simulink model "sfReuseStates"  (R2025b)
settings: Solver=FixedStepDiscrete  StartTime=0.0  StopTime=10.0  FixedStep=1  RelTol=1e-3  EnableMultiTasking=on
settings Model: Creator=The MathWorks, Inc.  LastModifiedBy=The MathWorks, Inc.
settings SolverCC: AlgebraicLoopSolver=TrustRegion
settings DataIOCC: LimitDataPoints=on  SaveFormat=Array  ReturnWorkspaceOutputs=off
settings OptimizationCC: ReuseModelBlockBuffer=off  ExpressionDepthLimit=2147483647.0  LifeSpan=1  EfficientTunableParamExpr=on
settings DebuggingCC: UnderspecifiedInitializationDetection=Classic  MergeDetectMultiDrivingBlocksExec=none  SolverPrmCheckMsg=warning  FcnCallInpInsideContextMsg=warning  UnconnectedInputMsg=warning  UnconnectedOutputMsg=warning  UnconnectedLineMsg=warning  StateNameClashWarn=warning  SFUnexpectedBacktrackingDiag=warning  SFNoUnconditionalDefaultTransitionDiag=warning  SFExecutionAtInitializationDiag=none  ArithmeticOperatorsInVariantConditions=warning
settings HardwareCC: ProdBitPerPointer=32.0  ProdBitPerSizeT=32.0  ProdBitPerPtrDiffT=32.0  ProdLargestAtomicFloat=None  ProdIntDivRoundTo=Undefined  ProdEndianess=Unspecified  ProdWordSize=32.0  ProdHWDeviceType=32-bit Generic
settings ModelReferenceCC: EnableRefExpFcnMdlSchedulingChecks=on  PropagateSignalLabelsOutOfModel=off
settings SFSimCC: SimUseLocalCustomCode=off  SimParseCustomCode=off  MATLABDynamicMemAlloc=off
settings RTWCC: SystemTargetFile=ert.tlc  TemplateMakefile=ert_default_tmf  GenerateReport=on  RTWUseLocalCustomCode=off  IncludeHyperlinkInReport=on  LaunchReport=on  GenerateTraceInfo=on  GenerateTraceReport=on  GenerateTraceReportSl=on  GenerateTraceReportSf=on  GenerateTraceReportEml=on  GPUComputeCapability=3.5  Description=Real-Time Workshop Embedded Coder
settings CodeAppCC: IgnoreCustomStorageClasses=off  CustomSymbolStrType=$N$R$M  StateflowObjectComments=on  InternalIdentifier=Classic
settings ERTTargetCC: InlinedParameterPlacement=Hierarchical  ERTCustomFileTemplate=example_file_process.tlc  ConvertIfToSwitch=off  SuppressUnreachableDefaultCases=off  MultiwordLength=2048.0  GenerateSampleERTMain=on  SupportContinuousTime=on
settings ConfigComp: CovMetricSettings=dw  CovSaveCumulativeToWorkspaceVar=on  CovSaveSingleToWorkspaceVar=on  CovExternalEMLEnable=off

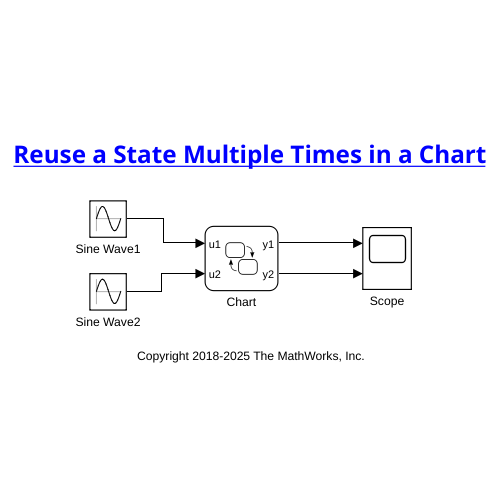
[thumbnail: Simulink's stored preview of the top-level diagram]
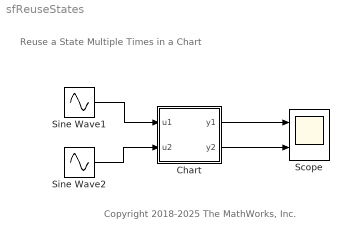
== system sfReuseStates ==
  note: Copyright 2018-2025 The MathWorks, Inc.
  note: Reuse a State Multiple Times in a Chart
  Chart : Stateflow chart  TreatAsAtomicUnit=on
  Scope : Scope  NumInputPorts=2
      settings: ActiveDisplayYMinimum=-5  ActiveDisplayYMaximum=5
  Sine Wave1 : Sin  SampleTime=0
  Sine Wave2 : Sin  Frequency=2  SampleTime=0
  wires:
  Chart/1(y1) -> Scope/1
  Chart/2(y2) -> Scope/2
  Sine Wave1/1 -> Chart/1(u1)
  Sine Wave2/1 -> Chart/2(u2)

== stateflow chart sfReuseStates/Chart ==
  state A [parallel]
    settings: executionOrder=1
    state Pos
      entry: y1 = 1;
    state Neg
      entry: y1 = -1;
    (default) -> A.Pos [order 1] : [u1 > 0]
    (default) -> A.Neg [order 2]
    A.Pos -> A.Neg : [u1 < 0]
    A.Neg -> A.Pos : [u1 > 0]
  state B [parallel]
    settings: executionOrder=2
    state Pos
      entry: y2 = 1;
    state Neg
      entry: y2 = -1;
    (default) -> B.Pos [order 1] : [u2 > 0]
    (default) -> B.Neg [order 2]
    B.Pos -> B.Neg : [u2 < 0]
    B.Neg -> B.Pos : [u2 > 0]
  data: u1 input; u2 input; y1 output double; y2 output double
